simulink model "modelo_furuta"  (R2026a)
settings: Solver=ode45  StopTime=8

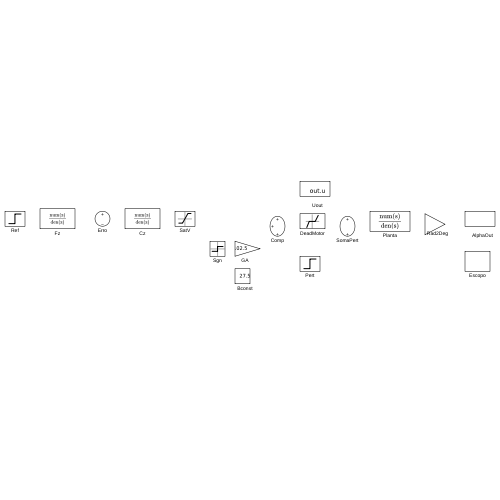
[thumbnail: Simulink's stored preview of the top-level diagram]
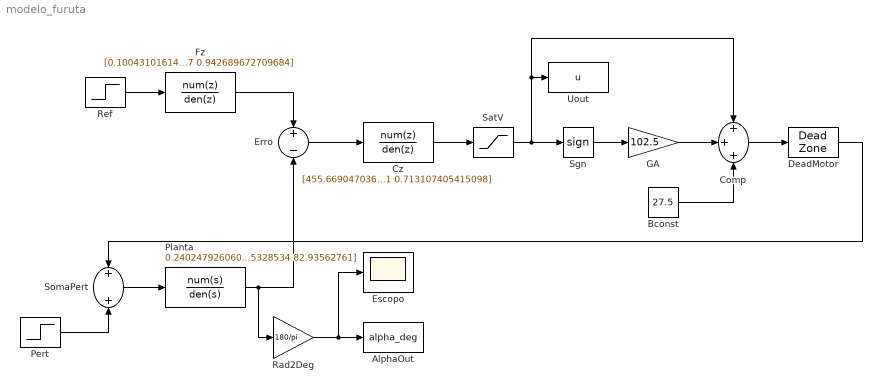
== system modelo_furuta ==
  AlphaOut : ToWorkspace  VariableName=alpha_deg  SaveFormat=Timeseries  SampleTime=-1
  Bconst : Constant  Value=27.5
  Comp : Sum  Inputs=+++
  Cz : DiscreteTransferFcn  Numerator=[455.669047036076 -881.983785427658 429.554504814372]  Denominator=[1 -1.7131074054151 0.713107405415098]  SampleTime=0.02
  DeadMotor : DeadZone  LowerValue=-75  UpperValue=130
  Erro : Sum  Inputs=+-
  Escopo : Scope
  Fz : DiscreteTransferFcn  Numerator=[0.100431016142942 -0.147266633553737 0.0539455285269075]  Denominator=[1 -1.93557976159357 0.942689672709684]  SampleTime=0.02
  GA : Gain  Gain=102.5
  Pert : Step  Time=2  FinalValue=40  SampleTime=0
  Planta : TransferFcn  Numerator=0.240247926060648  Denominator=[1 1.35328534 82.93562761]
  Rad2Deg : Gain  Gain=180/pi
  Ref : Step  Time=0  FinalValue=0  SampleTime=0
  SatV : Saturate  UpperLimit=255  LowerLimit=-255
  Sgn : Signum
  SomaPert : Sum
  Uout : ToWorkspace  VariableName=u  SaveFormat=Timeseries  SampleTime=-1
  wires:
  DeadMotor/1 -> SomaPert/1
  Pert/1 -> SomaPert/2
  Ref/1 -> Fz/1
  Fz/1 -> Erro/1
  Planta/1 -> Rad2Deg/1, Erro/2
  Bconst/1 -> Comp/3
  Rad2Deg/1 -> Escopo/1, AlphaOut/1
  Cz/1 -> SatV/1
  SatV/1 -> Uout/1, Comp/1, Sgn/1
  SomaPert/1 -> Planta/1
  Sgn/1 -> GA/1
  Erro/1 -> Cz/1
  GA/1 -> Comp/2
  Comp/1 -> DeadMotor/1
